simulink model "lqr_sim"  (R2024b)
settings: Solver=VariableStepAuto  StartTime=0.0  StopTime=200  RelTol=1e-3
values from neighbouring files (symbols this model uses):
  A = [0 1 0 0 ... (first row only)    [calculate_k.m]
  B = [0; 0.1; 0; 0]    [calculate_k.m]
  init = [0.2; 0; 0.5; 0]    [calculate_k.m]
undefined symbols (not defined in the file or in its folder): K_lqr
settings Model: Creator=eduar  LastModifiedBy=eduar

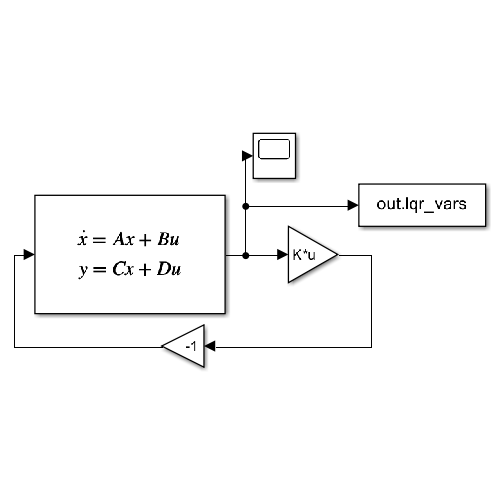
[thumbnail: Simulink's stored preview of the top-level diagram]
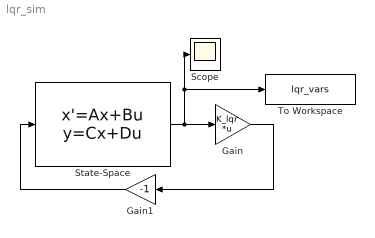
== system lqr_sim ==
  Gain : Gain  Gain=K_lqr  Multiplication=Matrix(K*u)
  Gain1 : Gain  Gain=-1
  Scope : Scope
  State-Space : StateSpace  A=A  B=B  C=eye(4)  D=zeros(4,1)  InitialCondition=init
  To Workspace : ToWorkspace  VariableName=lqr_vars  SaveFormat=Timeseries  SampleTime=-1
  wires:
  State-Space/1 -> To Workspace/1, Scope/1, Gain/1
  Gain1/1 -> State-Space/1
  Gain/1 -> Gain1/1
